simulink model "My_gfm_battery_sil_1_Exciter_1"  (R2018b)
settings: Solver=ode23t  StartTime=0.0  StopTime=30  MaxStep=1e-4  RelTol=1e-3
PreLoadFcn:
  | modelDir = fileparts(get_param(bdroot,'FileName'));
  | 
  | load_system(fullfile(modelDir,'controls_element_lib.slx'));
  | load_system(fullfile(modelDir,'test_sequence_lib.slx'));
InitFcn:
  | close all;
  | clear all;
  | clc;
  | 
  | % frequency nominals
  | F_NOM = 60;
  | W_NOM = 2 * pi * F_NOM;
  | 
  | % base values relative to inverter
  | % --------------------------------
  | VLL_INV_NOM = 480;
  | P_INV_NOM = 1e6;
  | Q_INV_NOM = 0.5e6;
  | S_INV_NOM = sqrt(P_INV_NOM^2 + Q_INV_NOM^2);
  | 
  | I_INV_BASE = S_INV_NOM/(sqrt(3)*VLL_INV_NOM);
  | Z_INV_BASE = VLL_INV_NOM^2/S_INV_NOM;
  | L_INV_BASE = Z_INV_BASE / W_NOM;
  | C_INV_BASE = 1 / (Z_INV_BASE * W_NOM);
  | 
  | % nominal ratings for power system model
  | % --------------------------------------
  | INVERTER_COUNT = 100;
  | 
  | VLV_NOM = VLL_INV_NOM;
  | VMV_NOM = 35e3;
  | VHV_NOM = 230e3;
  | S_PLANT = INVERTER_COUNT * S_INV_NOM;
  | 
  | N_GSU = VHV_NOM/VMV_NOM;
  | N_MVT = VMV_NOM/VLV_NOM;
  | 
  | I_LV_BASE = S_PLANT/(sqrt(3)*VLV_NOM);
  | I_MV_BASE = S_PLANT/(sqrt(3)*VMV_NOM);
  | I_HV_BASE = S_PLANT/(sqrt(3)*VHV_NOM);
  | 
  | Z_LV_BASE = VLV_NOM^2/S_PLANT;
  | Z_MV_BASE = VMV_NOM^2/S_PLANT;
  | Z_HV_BASE = VHV_NOM^2/S_PLANT;
  | 
  | L_LV_BASE = Z_LV_BASE / W_NOM;
  | L_MV_BASE = Z_MV_BASE / W_NOM;
  | L_HV_BASE = Z_HV_BASE / W_NOM;
  | C_LV_BASE = 1 / (Z_LV_BASE * W_NOM);
  | C_MV_BASE = 1 / (Z_MV_BASE * W_NOM);
  | C_HV_BASE = 1 / (Z_HV_BASE * W_NOM);
undefined symbols (not defined in the file): j
libraries: simulink x38, test_sequence_lib x10, controls_element_lib x9
(part 2 of 6)

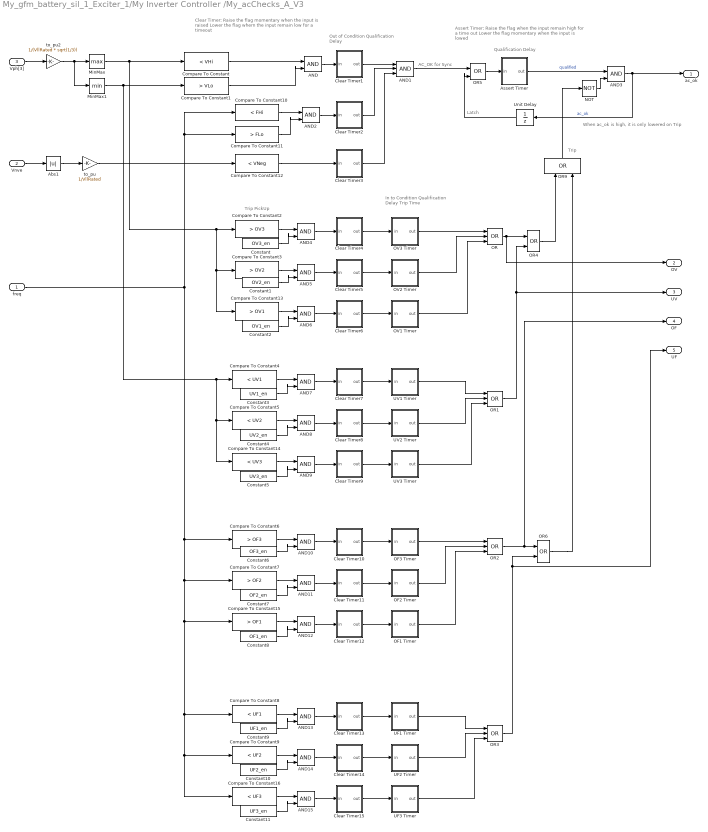
== system My_gfm_battery_sil_1_Exciter_1/My Inverter Controller /My_acChecks_A_V3 ==
  note: Trip
  note: Clear Timer:
      | Raise the flag momentary when the input is raised
      | Lower the flag whern the input remain low for a timeout
  note: AC_OK for Sync
  note: Assert Timer:
      | Raise the flag when the input remain high for a time out
      | Lower the flag momentary when the input is lowed
  note: Latch
  note: Qualification Delay
  note: When ac_ok is high, it is only lowered on Trip
  note: Out of Condition
      | Qualification Delay
  note: In to Condition
      | Qualification Delay
      | Trip Time
  note: Trip PickUp
  freq : Inport
  Vnve : Inport  Port=2
  Vph[3] : Inport  Port=3
  AND{,2..15} (15 alike) : Logic  IconShape=distinctive  AllPortsSameDT=off  OutDataTypeStr=boolean
  AND1 : Logic  Inputs=3  IconShape=distinctive  AllPortsSameDT=off  OutDataTypeStr=boolean
  Abs1 : Abs
  Assert Timer : Subsystem  mask{T_STEP=Ts, TIMEOUT=Time1}
      mask prompts: T_STEP "Time step"
  Clear Timer1 : Subsystem  mask{T_STEP=Ts, TIMEOUT=Time2, TIMER_INIT=0}
      mask prompts: T_STEP "Time step"; TIMER_INIT "Timer initial value"
  Clear Timer10 : Subsystem  mask{T_STEP=Ts, TIMEOUT=Time3, TIMER_INIT=0}
      mask prompts: T_STEP "Time step"; TIMER_INIT "Timer initial value"
  Clear Timer11 : Subsystem  mask{T_STEP=Ts, TIMEOUT=Time3, TIMER_INIT=0}
      mask prompts: T_STEP "Time step"; TIMER_INIT "Timer initial value"
  Clear Timer12 : Subsystem  mask{T_STEP=Ts, TIMEOUT=Time3, TIMER_INIT=0}
      mask prompts: T_STEP "Time step"; TIMER_INIT "Timer initial value"
  Clear Timer13 : Subsystem  mask{T_STEP=Ts, TIMEOUT=Time3, TIMER_INIT=0}
      mask prompts: T_STEP "Time step"; TIMER_INIT "Timer initial value"
  Clear Timer14 : Subsystem  mask{T_STEP=Ts, TIMEOUT=Time3, TIMER_INIT=0}
      mask prompts: T_STEP "Time step"; TIMER_INIT "Timer initial value"
  Clear Timer15 : Subsystem  mask{T_STEP=Ts, TIMEOUT=Time3, TIMER_INIT=0}
      mask prompts: T_STEP "Time step"; TIMER_INIT "Timer initial value"
  Clear Timer2 : Subsystem  mask{T_STEP=Ts, TIMEOUT=Time2, TIMER_INIT=0}
      mask prompts: T_STEP "Time step"; TIMER_INIT "Timer initial value"
  Clear Timer3 : Subsystem  mask{T_STEP=Ts, TIMEOUT=Time2, TIMER_INIT=0}
      mask prompts: T_STEP "Time step"; TIMER_INIT "Timer initial value"
  Clear Timer4 : Subsystem  mask{T_STEP=Ts, TIMEOUT=Time3, TIMER_INIT=0}
      mask prompts: T_STEP "Time step"; TIMER_INIT "Timer initial value"
  Clear Timer5 : Subsystem  mask{T_STEP=Ts, TIMEOUT=Time3, TIMER_INIT=0}
      mask prompts: T_STEP "Time step"; TIMER_INIT "Timer initial value"
  Clear Timer6 : Subsystem  mask{T_STEP=Ts, TIMEOUT=Time3, TIMER_INIT=0}
      mask prompts: T_STEP "Time step"; TIMER_INIT "Timer initial value"
  Clear Timer7 : Subsystem  mask{T_STEP=Ts, TIMEOUT=Time3, TIMER_INIT=0}
      mask prompts: T_STEP "Time step"; TIMER_INIT "Timer initial value"
  Clear Timer8 : Subsystem  mask{T_STEP=Ts, TIMEOUT=Time3, TIMER_INIT=0}
      mask prompts: T_STEP "Time step"; TIMER_INIT "Timer initial value"
  Clear Timer9 : Subsystem  mask{T_STEP=Ts, TIMEOUT=Time3, TIMER_INIT=0}
      mask prompts: T_STEP "Time step"; TIMER_INIT "Timer initial value"
  Compare To Constant : simulink/Logic and Bit Operations/Compare To Constant  relop=<  const=VHi  OutDataTypeStr=boolean
  Compare To Constant1 : simulink/Logic and Bit Operations/Compare To Constant  relop=>  const=VLo  OutDataTypeStr=boolean
  Compare To Constant10 : simulink/Logic and Bit Operations/Compare To Constant  relop=<  const=FHi  OutDataTypeStr=boolean
  Compare To Constant11 : simulink/Logic and Bit Operations/Compare To Constant  relop=>  const=FLo  OutDataTypeStr=boolean
  Compare To Constant12 : simulink/Logic and Bit Operations/Compare To Constant  relop=<  const=VNeg  OutDataTypeStr=boolean
  Compare To Constant13 : simulink/Logic and Bit Operations/Compare To Constant  relop=>  const=OV1  OutDataTypeStr=boolean
  Compare To Constant14 : simulink/Logic and Bit Operations/Compare To Constant  relop=<  const=UV3  OutDataTypeStr=boolean
  Compare To Constant15 : simulink/Logic and Bit Operations/Compare To Constant  relop=>  const=OF1  OutDataTypeStr=boolean
  Compare To Constant16 : simulink/Logic and Bit Operations/Compare To Constant  relop=<  const=UF3  OutDataTypeStr=boolean
  Compare To Constant2 : simulink/Logic and Bit Operations/Compare To Constant  relop=>  const=OV3  OutDataTypeStr=boolean
  Compare To Constant3 : simulink/Logic and Bit Operations/Compare To Constant  relop=>  const=OV2  OutDataTypeStr=boolean
  Compare To Constant4 : simulink/Logic and Bit Operations/Compare To Constant  relop=<  const=UV1  OutDataTypeStr=boolean
  Compare To Constant5 : simulink/Logic and Bit Operations/Compare To Constant  relop=<  const=UV2  OutDataTypeStr=boolean
  Compare To Constant6 : simulink/Logic and Bit Operations/Compare To Constant  relop=>  const=OF3  OutDataTypeStr=boolean
  Compare To Constant7 : simulink/Logic and Bit Operations/Compare To Constant  relop=>  const=OF2  OutDataTypeStr=boolean
  Compare To Constant8 : simulink/Logic and Bit Operations/Compare To Constant  relop=<  const=UF1  OutDataTypeStr=boolean
  Compare To Constant9 : simulink/Logic and Bit Operations/Compare To Constant  relop=<  const=UF2  OutDataTypeStr=boolean
  Constant : Constant  Value=OV3_en
  Constant1 : Constant  Value=OV2_en
  Constant10 : Constant  Value=UF2_en
  Constant11 : Constant  Value=UF3_en
  Constant2 : Constant  Value=OV1_en
  Constant3 : Constant  Value=UV1_en
  Constant4 : Constant  Value=UV2_en
  Constant5 : Constant  Value=UV3_en
  Constant6 : Constant  Value=OF3_en
  Constant7 : Constant  Value=OF2_en
  Constant8 : Constant  Value=OF1_en
  Constant9 : Constant  Value=UF1_en
  MinMax : MinMax  Function=max
  MinMax1 : MinMax
  NOT : Logic  Operator=NOT  IconShape=distinctive  AllPortsSameDT=off  OutDataTypeStr=boolean
  OF1 Timer : Subsystem  mask{T_STEP=Ts, TIMEOUT=OF1_Time}
      mask prompts: T_STEP "Time step"
  OF2 Timer : Subsystem  mask{T_STEP=Ts, TIMEOUT=OF2_Time}
      mask prompts: T_STEP "Time step"
  OF3 Timer : Subsystem  mask{T_STEP=Ts, TIMEOUT=OF3_Time}
      mask prompts: T_STEP "Time step"
  OR{,1..3} (4 alike) : Logic  Operator=OR  Inputs=3  IconShape=distinctive  AllPortsSameDT=off  OutDataTypeStr=boolean
  OR{4..6,9} (4 alike) : Logic  Operator=OR  IconShape=distinctive  AllPortsSameDT=off  OutDataTypeStr=boolean
  OV1 Timer : Subsystem  mask{T_STEP=Ts, TIMEOUT=OV1_Time}
      mask prompts: T_STEP "Time step"
  OV2 Timer : Subsystem  mask{T_STEP=Ts, TIMEOUT=OV2_Time}
      mask prompts: T_STEP "Time step"
  OV3 Timer : Subsystem  mask{T_STEP=Ts, TIMEOUT=OV3_Time}
      mask prompts: T_STEP "Time step"
  UF1 Timer : Subsystem  mask{T_STEP=Ts, TIMEOUT=UF1_Time}
      mask prompts: T_STEP "Time step"
  UF2 Timer : Subsystem  mask{T_STEP=Ts, TIMEOUT=UF2_Time}
      mask prompts: T_STEP "Time step"
  UF3 Timer : Subsystem  mask{T_STEP=Ts, TIMEOUT=UF3_Time}
      mask prompts: T_STEP "Time step"
  UV1 Timer : Subsystem  mask{T_STEP=Ts, TIMEOUT=UV1_Time}
      mask prompts: T_STEP "Time step"
  UV2 Timer : Subsystem  mask{T_STEP=Ts, TIMEOUT=UV2_Time}
      mask prompts: T_STEP "Time step"
  UV3 Timer : Subsystem  mask{T_STEP=Ts, TIMEOUT=UV3_Time}
      mask prompts: T_STEP "Time step"
  Unit Delay : UnitDelay  SampleTime=Ts
  to_pu : Gain  Gain=1/VllRated
  to_pu2 : Gain  Gain=1/(VllRated * sqrt(1/3))
  ac_ok : Outport  VectorParamsAs1DForOutWhenUnconnected=on
  OV : Outport  Port=2  VectorParamsAs1DForOutWhenUnconnected=on
  UV : Outport  Port=3  VectorParamsAs1DForOutWhenUnconnected=on
  OF : Outport  Port=4  VectorParamsAs1DForOutWhenUnconnected=on
  UF : Outport  Port=5  VectorParamsAs1DForOutWhenUnconnected=on
  wires:
  Vph[3]/1 -> to_pu2/1
  OR4/1 -> OR9/1
  OR9/1 -> NOT/1
  to_pu/1 -> Compare To Constant12/1
  MinMax/1 -> Compare To Constant13/1, Compare To Constant3/1, Compare To Constant2/1, Compare To Constant/1
  Abs1/1 -> to_pu/1
  Unit Delay/1 -> OR5/2
  OV3 Timer/1(out) -> OR/1
  Compare To Constant12/1 -> Clear Timer3/1(in)
  Clear Timer3/1(out) -> AND1/3
  Assert Timer/1(out) -> AND3/1  "qualified"
  UV2 Timer/1(out) -> OR1/2
  OF3 Timer/1(out) -> OR2/1
  Clear Timer10/1(out) -> OF3 Timer/1(in)
  Compare To Constant6/1 -> AND10/1
  Clear Timer11/1(out) -> OF2 Timer/1(in)
  Clear Timer4/1(out) -> OV3 Timer/1(in)
  UF1 Timer/1(out) -> OR3/1
  UF2 Timer/1(out) -> OR3/2
  Vnve/1 -> Abs1/1
  NOT/1 -> AND3/2
  UV1 Timer/1(out) -> OR1/1
  AND2/1 -> Clear Timer2/1(in)
  Compare To Constant11/1 -> AND2/2
  OF2 Timer/1(out) -> OR2/2
  Clear Timer7/1(out) -> UV1 Timer/1(in)
  OR1/1 -> UV/1, OR4/2
  Clear Timer13/1(out) -> UF1 Timer/1(in)
  Compare To Constant7/1 -> AND11/1
  Clear Timer2/1(out) -> AND1/2
  Clear Timer14/1(out) -> UF2 Timer/1(in)
  Clear Timer5/1(out) -> OV2 Timer/1(in)
  freq/1 -> Compare To Constant11/1, Compare To Constant10/1, Compare To Constant8/1, Compare To Constant16/1, Compare To Constant9/1, Compare To Constant15/1, Compare To Constant7/1, Compare To Constant6/1
  OV2 Timer/1(out) -> OR/2
  Compare To Constant10/1 -> AND2/1
  Clear Timer1/1(out) -> AND1/1
  OR/1 -> OV/1, OR4/1
  Clear Timer8/1(out) -> UV2 Timer/1(in)
  AND3/1 -> ac_ok/1, Unit Delay/1  "ac_ok"
  Compare To Constant2/1 -> AND4/1
  Compare To Constant3/1 -> AND5/1
  AND/1 -> Clear Timer1/1(in)
  Compare To Constant/1 -> AND/1
  Compare To Constant1/1 -> AND/2
  AND1/1 -> OR5/1
  OR5/1 -> Assert Timer/1(in)
  to_pu2/1 -> MinMax1/1, MinMax/1
  Clear Timer6/1(out) -> OV1 Timer/1(in)
  OV1 Timer/1(out) -> OR/3
  Clear Timer9/1(out) -> UV3 Timer/1(in)
  UV3 Timer/1(out) -> OR1/3
  MinMax1/1 -> Compare To Constant4/1, Compare To Constant14/1, Compare To Constant5/1, Compare To Constant1/1
  Compare To Constant15/1 -> AND12/1
  OF1 Timer/1(out) -> OR2/3
  Clear Timer12/1(out) -> OF1 Timer/1(in)
  Clear Timer15/1(out) -> UF3 Timer/1(in)
  UF3 Timer/1(out) -> OR3/3
  AND4/1 -> Clear Timer4/1(in)
  Constant/1 -> AND4/2
  AND5/1 -> Clear Timer5/1(in)
  Constant1/1 -> AND5/2
  Compare To Constant13/1 -> AND6/1
  AND6/1 -> Clear Timer6/1(in)
  Constant2/1 -> AND6/2
  Compare To Constant4/1 -> AND7/1
  AND7/1 -> Clear Timer7/1(in)
  Compare To Constant5/1 -> AND8/1
  AND8/1 -> Clear Timer8/1(in)
  Compare To Constant14/1 -> AND9/1
  AND9/1 -> Clear Timer9/1(in)
  Constant3/1 -> AND7/2
  Constant4/1 -> AND8/2
  Constant5/1 -> AND9/2
  AND10/1 -> Clear Timer10/1(in)
  AND11/1 -> Clear Timer11/1(in)
  AND12/1 -> Clear Timer12/1(in)
  Constant6/1 -> AND10/2
  Constant7/1 -> AND11/2
  Constant8/1 -> AND12/2
  Compare To Constant8/1 -> AND13/1
  Constant9/1 -> AND13/2
  Compare To Constant9/1 -> AND14/1
  Constant10/1 -> AND14/2
  AND13/1 -> Clear Timer13/1(in)
  AND14/1 -> Clear Timer14/1(in)
  AND15/1 -> Clear Timer15/1(in)
  Compare To Constant16/1 -> AND15/1
  Constant11/1 -> AND15/2
  OR2/1 -> OF/1, OR6/1
  OR3/1 -> OR6/2, UF/1
  OR6/1 -> OR9/2

== system My_gfm_battery_sil_1_Exciter_1/My Inverter Controller /My_acMonitor_A ==
  note: Remove the second order ripple, dc value is RMS
  note: RMS LL Pos Seq Voltage (Vd+, Vq+)
  note: RMS LL Neg Seq Voltage (Vd-, Vq-)
  note: cos x + j sin x
      | cos (x-120) + j (sin x -120)
      | cos (x+120) + j (sin x +120)
  note: Hz
  note: RMS Va, Vb, Vc
  v_ac : Inport
  Analyzer_V : Subsystem
  Analyzer_V1 : Subsystem  Commented=on
  Gain2 : Gain  Gain=2
  PLL_3ph : Subsystem
  RMS_Analyzer : Subsystem
  SOGI : Subsystem
  Scope : Scope  NumInputPorts=3
  Scope1 : Scope  NumInputPorts=4
  Scope2 : Scope  NumInputPorts=2
  Terminator : Terminator
  to_pu : Gain  Gain=1/VllRated
  pll_freq : Outport  VectorParamsAs1DForOutWhenUnconnected=on
  pll_osc[3] : Outport  Port=2  VectorParamsAs1DForOutWhenUnconnected=on
  Vpve : Outport  Port=3  VectorParamsAs1DForOutWhenUnconnected=on
  Vnve : Outport  Port=4  VectorParamsAs1DForOutWhenUnconnected=on
  Vph[3] : Outport  Port=5  VectorParamsAs1DForOutWhenUnconnected=on
  wires:
  SOGI/1(notch) -> Scope/3, Vph[3]/1
  Gain2/1 -> SOGI/2(fnom)
  RMS_Analyzer/1(RMS) -> Scope/2, SOGI/1(in)
  Analyzer_V/4(Nve) -> Scope1/4, Vnve/1
  Analyzer_V/3(Pve) -> Vpve/1, Scope1/3
  PLL_3ph/1(osc[3]) -> pll_osc[3]/1, Scope2/2, Analyzer_V/2(osc[3])
  PLL_3ph/2(freq) -> Gain2/1, pll_freq/1
  v_ac/1 -> to_pu/1, Analyzer_V/1(in[3]), Scope/1, RMS_Analyzer/1(in)
  to_pu/1 -> Scope2/1, PLL_3ph/1(ref)
  Analyzer_V/1(fund[3]) -> Scope1/1
  Analyzer_V/2(Zero) -> Scope1/2
  SOGI/2(bpf) -> Terminator/1

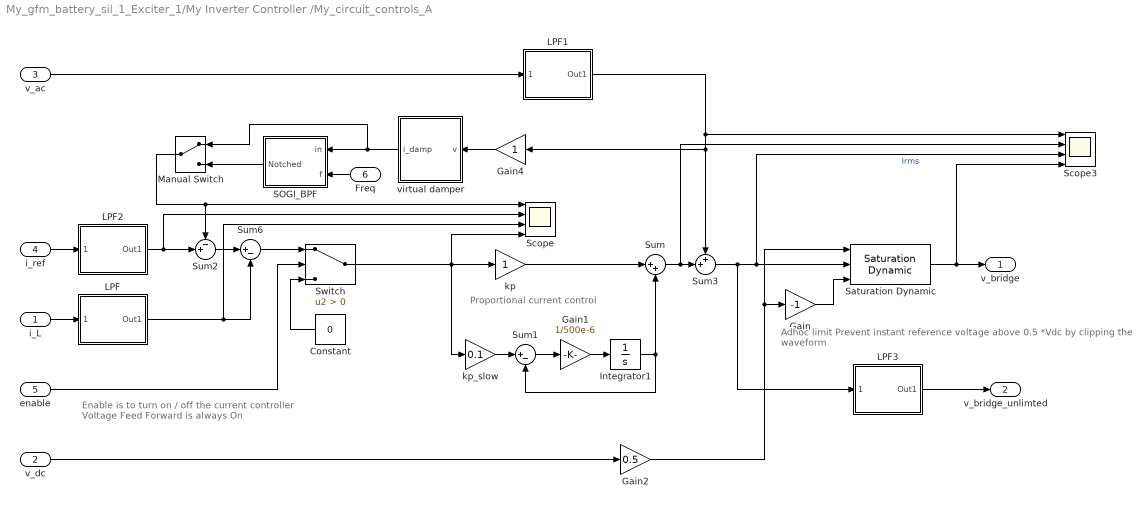
== system My_gfm_battery_sil_1_Exciter_1/My Inverter Controller /My_circuit_controls_A ==
  note: Proportional current control
  note: Adhoc limit
      | Prevent instant reference voltage above 0.5 *Vdc by clipping the waveform
  note: Enable is to turn on / off the current controller
      | Voltage Feed Forward is always On
  i_L : Inport
  v_dc : Inport  Port=2
  v_ac : Inport  Port=3
  i_ref : Inport  Port=4
  enable : Inport  Port=5
  Freq : Inport  Port=6
  Constant : Constant  Value=0
  Gain : Gain  Gain=-1
  Gain1 : Gain  Gain=1/500e-6
  Gain2 : Gain  Gain=0.5
  Gain4 : Gain
  Integrator1 : Integrator
  LPF : Subsystem
  LPF1 : Subsystem
  LPF2 : Subsystem
  LPF3 : Subsystem
  Manual Switch : ManualSwitch
  SOGI_BPF : Subsystem
  Saturation Dynamic : simulink/Discontinuities/Saturation Dynamic  OutMin=[]  OutMax=[]  OutDataTypeStr=Inherit: Same as second input  OutDataType=fixdt(1, 16)  OutScaling=2^-10  DoSatur=off
  Scope : Scope  NumInputPorts=4
  Scope3 : Scope  NumInputPorts=4
  Sum : Sum  Inputs=|++
  Sum1 : Sum  Inputs=|+-
  Sum2 : Sum  Inputs=-+|
  Sum3 : Sum  Inputs=++|
  Sum6 : Sum  Inputs=|+-
  Switch : Switch  Criteria=u2 > Threshold
  kp : Gain
  kp_slow : Gain  Gain=0.1
  virtual damper : Subsystem
  v_bridge : Outport  VectorParamsAs1DForOutWhenUnconnected=on
  v_bridge_unlimted : Outport  Port=2  VectorParamsAs1DForOutWhenUnconnected=on
  wires:
  LPF1/1(Out1) -> Gain4/1, Sum3/1, Scope3/1
  LPF/1(Out1) -> Scope/3, Sum6/2
  Gain2/1 -> Gain/1, Saturation Dynamic/1
  v_ac/1 -> LPF1/1(1)
  enable/1 -> Switch/2
  Constant/1 -> Switch/3
  Sum6/1 -> Switch/1
  i_ref/1 -> LPF2/1(1)
  i_L/1 -> LPF/1(1)
  Saturation Dynamic/1 -> Scope3/4, v_bridge/1
  Sum/1 -> Scope3/2, Sum3/2
  Sum2/1 -> Sum6/1
  kp/1 -> Sum/1
  Integrator1/1 -> Sum/2, Sum1/2
  Sum1/1 -> Gain1/1
  Gain1/1 -> Integrator1/1
  kp_slow/1 -> Sum1/1
  v_dc/1 -> Gain2/1
  Gain/1 -> Saturation Dynamic/3
  LPF2/1(Out1) -> Scope/2, Sum2/2
  Switch/1 -> Scope/4, kp/1, kp_slow/1
  Gain4/1 -> virtual damper/1(v)
  Freq/1 -> SOGI_BPF/2(f)
  virtual damper/1(i_damp) -> Manual Switch/1, SOGI_BPF/1(in)
  Manual Switch/1 -> Scope/1, Sum2/1
  SOGI_BPF/1(Notched) -> Manual Switch/2
  Sum3/1 -> LPF3/1(1), Scope3/3, Saturation Dynamic/2  "Irms"
  LPF3/1(Out1) -> v_bridge_unlimted/1

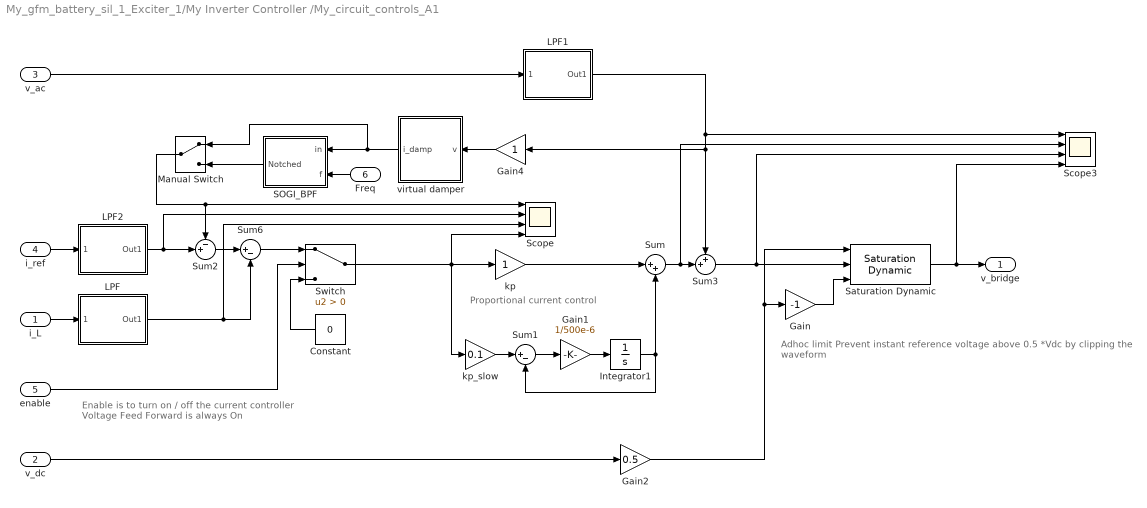
== system My_gfm_battery_sil_1_Exciter_1/My Inverter Controller /My_circuit_controls_A1 ==
  note: Proportional current control
  note: Adhoc limit
      | Prevent instant reference voltage above 0.5 *Vdc by clipping the waveform
  note: Enable is to turn on / off the current controller
      | Voltage Feed Forward is always On
  i_L : Inport
  v_dc : Inport  Port=2
  v_ac : Inport  Port=3
  i_ref : Inport  Port=4
  enable : Inport  Port=5
  Freq : Inport  Port=6
  Constant : Constant  Value=0
  Gain : Gain  Gain=-1
  Gain1 : Gain  Gain=1/500e-6
  Gain2 : Gain  Gain=0.5
  Gain4 : Gain
  Integrator1 : Integrator
  LPF : Subsystem
  LPF1 : Subsystem
  LPF2 : Subsystem
  Manual Switch : ManualSwitch
  SOGI_BPF : Subsystem
  Saturation Dynamic : simulink/Discontinuities/Saturation Dynamic  OutMin=[]  OutMax=[]  OutDataTypeStr=Inherit: Same as second input  OutDataType=fixdt(1, 16)  OutScaling=2^-10  DoSatur=off
  Scope : Scope  NumInputPorts=4
  Scope3 : Scope  NumInputPorts=4
  Sum : Sum  Inputs=|++
  Sum1 : Sum  Inputs=|+-
  Sum2 : Sum  Inputs=-+|
  Sum3 : Sum  Inputs=++|
  Sum6 : Sum  Inputs=|+-
  Switch : Switch  Criteria=u2 > Threshold
  kp : Gain
  kp_slow : Gain  Gain=0.1
  virtual damper : Subsystem
  v_bridge : Outport  VectorParamsAs1DForOutWhenUnconnected=on
  wires:
  LPF1/1(Out1) -> Gain4/1, Sum3/1, Scope3/1
  LPF/1(Out1) -> Scope/3, Sum6/2
  Gain2/1 -> Gain/1, Saturation Dynamic/1
  v_ac/1 -> LPF1/1(1)
  enable/1 -> Switch/2
  Constant/1 -> Switch/3
  Sum6/1 -> Switch/1
  Sum3/1 -> Scope3/3, Saturation Dynamic/2
  i_ref/1 -> LPF2/1(1)
  i_L/1 -> LPF/1(1)
  Saturation Dynamic/1 -> Scope3/4, v_bridge/1
  Sum/1 -> Scope3/2, Sum3/2
  Sum2/1 -> Sum6/1
  kp/1 -> Sum/1
  Integrator1/1 -> Sum/2, Sum1/2
  Sum1/1 -> Gain1/1
  Gain1/1 -> Integrator1/1
  kp_slow/1 -> Sum1/1
  v_dc/1 -> Gain2/1
  Gain/1 -> Saturation Dynamic/3
  LPF2/1(Out1) -> Scope/2, Sum2/2
  Switch/1 -> Scope/4, kp/1, kp_slow/1
  Gain4/1 -> virtual damper/1(v)
  Freq/1 -> SOGI_BPF/2(f)
  virtual damper/1(i_damp) -> Manual Switch/1, SOGI_BPF/1(in)
  Manual Switch/1 -> Scope/1, Sum2/1
  SOGI_BPF/1(Notched) -> Manual Switch/2

== system My_gfm_battery_sil_1_Exciter_1/My Inverter Controller /My_currentLimiting_B ==
  note: LL RMS
  note: SOGI gain is 1 not 1/sqrt(2),
      | improve tracking over transients
  note: Only capture 60Hz component
  note: Iabc rms
  note: Peak_Iabc
  note: Only apply limit on 60 Hz components
  note: LL RMS
  Irms_limit : Inport
  freq : Inport  Port=2
  iref : Inport  Port=3
  v_bridge_unlimted : Inport  Port=4
  v_dc : Inport  Port=5
  Constant1 : Constant
  Current_foldback1 : Subsystem
  Gain1 : Gain  Gain=sqrt(3/2)
  Gain2 : Gain  Gain=0.5
  Gain3 : Gain  Gain=sqrt(3)
  Manual Switch : ManualSwitch  CurrentSetting=0
  Product : Product
  Product1 : Product
  RMS_Analyzer : Subsystem
  RMS_Analyzer1 : Subsystem
  SOGI_BPF : Subsystem
  Scope1 : Scope  NumInputPorts=3
  Scope11 : Scope  NumInputPorts=3
  Scope3 : Scope  NumInputPorts=3
  Sum1 : Sum  Inputs=|+-
  estimate_excess : Subsystem
  soft_saturation : Subsystem  mask{soft_limit=peakSoftLimit*IRated, hard_limit=peakHardLimit*IRated, Xau=1}
      mask prompts: soft_limit "Soft limit"; hard_limit "Hard limit"; Xau "Saturation Rate"
  soft_saturation1 : Subsystem  Commented=on  mask{soft_limit=peakSoftLimit*IRated, hard_limit=peakHardLimit*IRated}
      mask prompts: soft_limit "Soft limit"; hard_limit "Hard limit"
  to_pu : Gain  Gain=1/VLL_INV_NOM
  to_pu1 : Gain  Gain=1/VLL_INV_NOM
  iref_limited : Outport  VectorParamsAs1DForOutWhenUnconnected=on
  wires:
  soft_saturation/1(out) -> Scope3/2, Product/1
  estimate_excess/1(excess_fraction) -> Scope11/1, Product1/1
  RMS_Analyzer/1(RMS) -> estimate_excess/2(I[3])  "Irms"
  Product1/1 -> Scope11/3, Sum1/2  "i_excess"
  SOGI_BPF/1(bpf) -> Product1/2, Scope11/2
  freq/1 -> SOGI_BPF/2(f)
  iref/1 -> Sum1/1, RMS_Analyzer/1(in), SOGI_BPF/1(in)
  Irms_limit/1 -> estimate_excess/1(Ilimit)
  v_bridge_unlimted/1 -> RMS_Analyzer1/1(in)
  Sum1/1 -> soft_saturation/1(in)
  RMS_Analyzer1/1(RMS) -> Gain3/1
  v_dc/1 -> Gain2/1
  Gain2/1 -> Gain1/1
  to_pu/1 -> Current_foldback1/1(V[3]_pu), Scope1/2
  Gain3/1 -> to_pu/1
  to_pu1/1 -> Current_foldback1/2(Vmax), Scope1/3
  Product/1 -> Scope3/1, iref_limited/1
  Manual Switch/1 -> Product/2, Scope3/3
  Current_foldback1/1(limit_pu) -> Scope1/1, Manual Switch/2
  Constant1/1 -> Manual Switch/1
  Gain1/1 -> to_pu1/1

== system My_gfm_battery_sil_1_Exciter_1/My Inverter Controller /My_currentLimiting_B1 ==
  note: SOGI gain is 1 not 1/sqrt(2),
      | improve tracking over transients
  note: Only capture 60Hz component
  note: Iabc rms
  note: Peak_Iabc
  note: Only apply limit on 60 Hz components
  Irms_limit : Inport
  freq : Inport  Port=2
  iref : Inport  Port=3
  Product1 : Product
  RMS_Analyzer : Subsystem
  SOGI_BPF : Subsystem
  Scope11 : Scope  NumInputPorts=3
  Sum1 : Sum  Inputs=|+-
  estimate_excess : Subsystem
  soft_saturation : Subsystem  mask{soft_limit=peakSoftLimit*IRated, hard_limit=peakHardLimit*IRated, Xau=1}
      mask prompts: soft_limit "Soft limit"; hard_limit "Hard limit"; Xau "Saturation Rate"
  soft_saturation1 : Subsystem  Commented=on  mask{soft_limit=peakSoftLimit*IRated, hard_limit=peakHardLimit*IRated}
      mask prompts: soft_limit "Soft limit"; hard_limit "Hard limit"
  iref_limited : Outport  VectorParamsAs1DForOutWhenUnconnected=on
  wires:
  soft_saturation/1(out) -> iref_limited/1
  estimate_excess/1(excess_fraction) -> Scope11/1, Product1/1
  RMS_Analyzer/1(RMS) -> estimate_excess/2(I[3])  "Irms"
  Product1/1 -> Scope11/3, Sum1/2  "i_excess"
  Sum1/1 -> soft_saturation/1(in)
  SOGI_BPF/1(bpf) -> Product1/2, Scope11/2
  freq/1 -> SOGI_BPF/2(f)
  iref/1 -> Sum1/1, RMS_Analyzer/1(in), SOGI_BPF/1(in)
  Irms_limit/1 -> estimate_excess/1(Ilimit)

== system My_gfm_battery_sil_1_Exciter_1/My Inverter Controller /My_currentSource_A ==
  note: S = sqrt(3)*V *conj(I)
      | P+jQ = sqrt(3)*(vd+jvq)*(id-jiq)
      | so P-jQ = sqrt(3)*(vd-jvq)*(id+jiq)
      | vq = 0, vd is LL RMS, id,iq are RMS
  note: S = sqrt(3) * VLL_rms * Irms
  note: RMS Id, Iq
  note: Vd+
  note: Why?
  note: RMS LL Pos Seq Voltage (Vd+, Vq+)
  note: Peak_Iabc
  note: cos x + j sin x
      | cos (x-120) + j (sin x -120)
      | cos (x+120) + j (sin x +120)
  enable : Inport
  P_request : Inport  Port=2
  Q_request : Inport  Port=3
  osc : Inport  Port=4
  Vpve : Inport  Port=5
  AND4 : Logic  IconShape=distinctive  AllPortsSameDT=off  OutDataTypeStr=boolean
  Complex to Real-Imag : ComplexToRealImag
  Conj : Math  Operator=conj  SaturateOnIntegerOverflow=on
  Constant : Constant  Value=0
  Constant2 : Constant  Value=CSOnline
  Divide : Product  Inputs=*/
  Gain : Gain  Gain=1/sqrt(3)
  Max1 : MinMax  Function=max  Inputs=2
  Real-Imag to Complex : RealImagToComplex
  Scope : Scope
  Switch : Switch  Criteria=u2 > Threshold
  Terminator : Terminator
  VLL_RATED : Constant  Value=VllRated
  current_modulator : Subsystem
  iref : Outport  VectorParamsAs1DForOutWhenUnconnected=on
  wires:
  Q_request/1 -> Real-Imag to Complex/2
  P_request/1 -> Real-Imag to Complex/1
  Complex to Real-Imag/1 -> Max1/1
  VLL_RATED/1 -> Max1/2
  Max1/1 -> Divide/2
  Divide/1 -> Gain/1
  Vpve/1 -> Complex to Real-Imag/1
  current_modulator/1(i_ref) -> Switch/1
  osc/1 -> current_modulator/2(osc)
  Real-Imag to Complex/1 -> Conj/1
  Conj/1 -> Divide/1
  Gain/1 -> Scope/1, current_modulator/1(I_cmd)
  Complex to Real-Imag/2 -> Terminator/1
  Constant/1 -> Switch/3
  Switch/1 -> iref/1
  Constant2/1 -> AND4/2
  AND4/1 -> Switch/2
  enable/1 -> AND4/1

== system My_gfm_battery_sil_1_Exciter_1/My Inverter Controller /My_machineModel_A ==
  note: Assume circuit controls will achieve
      | Iref = Imeas in the freq range of interest
  note: Measured terminal voltage
  note: Aligning with Rotor Frame
      | cos x + j sin x
      | cos (x-120) + j (sin x -120)
      | cos (x+120) + j (sin x +120)
  note: Peak Va, Vb, Vc
  note: RMS LL Vd
  note: RMS LL Vq
  Vref : Inport
  Prequest : Inport  Port=2
  Ex_Fref : Inport  Port=3
  PLL_Fref : Inport  Port=4
  v_terminal : Inport  Port=5
  enable : Inport  Port=6
  AND4 : Logic  IconShape=distinctive  AllPortsSameDT=off  OutDataTypeStr=boolean
  AVR : Subsystem  AncestorBlock=controls_element_lib/machineModel_A/excitation
  Constant1 : Constant  Value=FreqRefSel
  Constant2 : Constant  Value=MachOnline
  Exciter : Subsystem  AncestorBlock=controls_element_lib/machineModel_A/excitation
  Scope : Scope  NumInputPorts=3
  Scope1 : Scope  NumInputPorts=4
  Scope2 : Scope  NumInputPorts=4
  Switch : Switch  Criteria=u2 > Threshold
  governer : Subsystem
  impedance emulation : Subsystem
  power analyzer : Subsystem
  rotor model : Subsystem
  voltage analyzer : Subsystem
  rotor_freq : Outport  VectorParamsAs1DForOutWhenUnconnected=on
  iref : Outport  Port=2  VectorParamsAs1DForOutWhenUnconnected=on
  wires:
  Vref/1 -> AVR/1(VRef)
  Switch/1 -> governer/2(Fref)
  AND4/1 -> governer/3(enabled), AVR/3(enabled), impedance emulation/2(enable)
  voltage analyzer/1(Vd) -> Scope2/2, AVR/6(Vd)
  rotor model/2(f_rotor) -> Scope1/4, governer/6(f_rotor), Scope/1, rotor_freq/1  "f_rotor"
  voltage analyzer/2(Vq) -> governer/5(Vq), Scope2/3, AVR/7(Vq)
  v_terminal/1 -> Scope2/1, voltage analyzer/2(v_terminal), power analyzer/2(vac), Scope/3, impedance emulation/3(v_terminal)
  impedance emulation/1(i_ref) -> iref/1, AVR/5(iac), power analyzer/1(iac)
  Prequest/1 -> governer/1(Prequest)
  governer/1(power) -> Scope1/1, rotor model/1(p_mechanical)
  Exciter/1(v_emf) -> Scope/2, impedance emulation/1(v_emf)  "v_emf"
  power analyzer/1(P) -> Scope1/2, rotor model/2(p_electrical)  "p_electrical"
  rotor model/1(osc[3]) -> voltage analyzer/1(osc[3]), Exciter/2(osc[3]), AVR/4(osc[3])
  power analyzer/2(Q) -> Scope1/3, AVR/2(Q)
  voltage analyzer/3(Vt_Mag) -> governer/4(Vt), Scope2/4
  Constant1/1 -> Switch/2
  Ex_Fref/1 -> Switch/1
  PLL_Fref/1 -> Switch/3
  Constant2/1 -> AND4/2
  enable/1 -> AND4/1
  AVR/1(Vexc) -> Exciter/1(Vexc)

== system My_gfm_battery_sil_1_Exciter_1/My Inverter Controller /My_machineModel_A1 ==
  note: Assume circuit controls will achieve
      | Iref = Imeas in the freq range of interest
  note: Measured terminal voltage
  note: Aligning with Rotor Frame
      | cos x + j sin x
      | cos (x-120) + j (sin x -120)
      | cos (x+120) + j (sin x +120)
  note: Peak Va, Vb, Vc
  note: RMS LL Vd
  note: RMS LL Vq
  Vref : Inport
  Prequest : Inport  Port=2
  Ex_Fref : Inport  Port=3
  PLL_Fref : Inport  Port=4
  v_terminal : Inport  Port=5
  enable : Inport  Port=6
  AND4 : Logic  IconShape=distinctive  AllPortsSameDT=off  OutDataTypeStr=boolean
  Constant1 : Constant  Value=FreqRefSel
  Constant2 : Constant  Value=MachOnline
  Scope : Scope  NumInputPorts=3
  Scope1 : Scope  NumInputPorts=4
  Scope2 : Scope  NumInputPorts=4
  Switch : Switch  Criteria=u2 > Threshold
  Terminator : Terminator
  excitation : Subsystem  AncestorBlock=controls_element_lib/machineModel_A/excitation
  governer : Subsystem
  governer1 : Subsystem  Commented=on
  impedance emulation : Subsystem
  power analyzer : Subsystem
  rotor model : Subsystem
  voltage analyzer : Subsystem
  rotor_freq : Outport  VectorParamsAs1DForOutWhenUnconnected=on
  iref : Outport  Port=2  VectorParamsAs1DForOutWhenUnconnected=on
  wires:
  Vref/1 -> excitation/1(VRef)
  Switch/1 -> governer/2(Fref)
  AND4/1 -> governer/3(enabled), impedance emulation/2(enable)
  voltage analyzer/1(Vd) -> Scope2/2
  rotor model/2(f_rotor) -> Scope1/4, governer/6(f_rotor), Scope/1, rotor_freq/1  "f_rotor"
  voltage analyzer/2(Vq) -> governer/5(Vq), Scope2/3
  v_terminal/1 -> Scope2/1, voltage analyzer/2(v_terminal), power analyzer/2(vac), Scope/3, impedance emulation/3(v_terminal)
  impedance emulation/1(i_ref) -> iref/1, power analyzer/1(iac)
  Prequest/1 -> governer/1(Prequest)
  governer/1(power) -> Scope1/1, rotor model/1(p_mechanical)
  excitation/1(v_emf) -> Scope/2, impedance emulation/1(v_emf)  "v_emf"
  power analyzer/1(P) -> Scope1/2, rotor model/2(p_electrical)  "p_electrical"
  rotor model/1(osc[3]) -> excitation/2(osc[3]), voltage analyzer/1(osc[3])
  power analyzer/2(Q) -> Scope1/3, Terminator/1
  voltage analyzer/3(Vt_Mag) -> excitation/3(Vt), governer/4(Vt), Scope2/4
  Constant1/1 -> Switch/2
  Ex_Fref/1 -> Switch/1
  PLL_Fref/1 -> Switch/3
  Constant2/1 -> AND4/2
  enable/1 -> AND4/1

== system My_gfm_battery_sil_1_Exciter_1/My Inverter Controller /My_machineModel_Other Exciter ==
  note: Assume circuit controls will achieve
      | Iref = Imeas in the freq range of interest
  note: Measured terminal voltage
  note: Aligning with Rotor Frame
      | cos x + j sin x
      | cos (x-120) + j (sin x -120)
      | cos (x+120) + j (sin x +120)
  note: Peak Va, Vb, Vc
  note: RMS LL Vd
  note: RMS LL Vq
  Ex_Vref : Inport
  Prequest : Inport  Port=2
  Ex_Fref : Inport  Port=3
  PLL_Fref : Inport  Port=4
  v_terminal : Inport  Port=5
  enable : Inport  Port=6
  AND4 : Logic  IconShape=distinctive  AllPortsSameDT=off  OutDataTypeStr=boolean
  AVR : Subsystem  AncestorBlock=controls_element_lib/machineModel_A/excitation
  Constant1 : Constant  Value=FreqRefSel
  Constant2 : Constant  Value=MachOnline
  Exciter : Subsystem  AncestorBlock=controls_element_lib/machineModel_A/excitation
  Scope : Scope  NumInputPorts=3
  Scope1 : Scope  NumInputPorts=4
  Scope2 : Scope  NumInputPorts=4
  Switch : Switch  Criteria=u2 > Threshold
  governer : Subsystem
  impedance emulation : Subsystem
  power analyzer : Subsystem
  rotor model : Subsystem
  voltage analyzer : Subsystem
  rotor_freq : Outport  VectorParamsAs1DForOutWhenUnconnected=on
  iref : Outport  Port=2  VectorParamsAs1DForOutWhenUnconnected=on
  wires:
  Switch/1 -> governer/2(Fref)
  AND4/1 -> governer/3(enabled), impedance emulation/2(enable)
  voltage analyzer/1(Vd) -> AVR/2(Vt), Scope2/2
  rotor model/2(f_rotor) -> Scope1/4, governer/6(f_rotor), Scope/1, rotor_freq/1  "f_rotor"
  voltage analyzer/2(Vq) -> governer/5(Vq), Scope2/3
  v_terminal/1 -> Scope2/1, voltage analyzer/2(v_terminal), power analyzer/2(vac), Scope/3, impedance emulation/3(v_terminal)
  impedance emulation/1(i_ref) -> iref/1, power analyzer/1(iac)
  Prequest/1 -> governer/1(Prequest)
  governer/1(power) -> Scope1/1, rotor model/1(p_mechanical)
  Exciter/1(v_emf) -> Scope/2, impedance emulation/1(v_emf)  "v_emf"
  power analyzer/1(P) -> Scope1/2, rotor model/2(p_electrical)  "p_electrical"
  rotor model/1(osc[3]) -> voltage analyzer/1(osc[3]), Exciter/2(osc[3])
  power analyzer/2(Q) -> AVR/3(Q), Scope1/3
  voltage analyzer/3(Vt_Mag) -> governer/4(Vt), Scope2/4
  Constant1/1 -> Switch/2
  Ex_Fref/1 -> Switch/1
  PLL_Fref/1 -> Switch/3
  Constant2/1 -> AND4/2
  enable/1 -> AND4/1
  AVR/1(Vexc) -> Exciter/1(Vexc)
  Ex_Vref/1 -> AVR/1(VRef)

== system My_gfm_battery_sil_1_Exciter_1/My Inverter Controller /My_powerLimiter_A ==
  note: Why not using Vpve
  note: RMS_Id
  note: Peak_Iabc
  note: Power Limits from Battery Management system
  note: Ref current (Machine + Current source)
  note: cos x + j sin x
      | cos (x-120) + j (sin x -120)
      | cos (x+120) + j (sin x +120)
  i_ac : Inport
  v_ac : Inport  Port=2
  osc : Inport  Port=3
  P_lim_high : Inport  Port=4
  P_lim_low : Inport  Port=5
  Gain1 : Gain  Gain=1/(VllRated * sqrt(3))
  Product : Product
  Saturation Dynamic : simulink/Discontinuities/Saturation Dynamic  OutMin=[]  OutMax=[]  OutDataTypeStr=Inherit: Same as second input  OutDataType=fixdt(1, 16)  OutScaling=2^-10  DoSatur=off
  Sum of Elements : Sum  Inputs=+
  Sum1 : Sum  Inputs=|+-
  Transfer Fcn : TransferFcn  Denominator=[1/wPowerLimiter, 1]
  current_modulator : controls_element_lib/currentSource_A/current_modulator  SystemSampleTime=-1
  i_excess : Outport  VectorParamsAs1DForOutWhenUnconnected=on
  wires:
  Transfer Fcn/1 -> Sum1/1, Saturation Dynamic/2  "P_lpf"
  current_modulator/1 -> i_excess/1
  Saturation Dynamic/1 -> Sum1/2
  P_lim_low/1 -> Saturation Dynamic/3
  P_lim_high/1 -> Saturation Dynamic/1
  Sum1/1 -> Gain1/1
  Sum of Elements/1 -> Transfer Fcn/1  "P_inst"
  Gain1/1 -> current_modulator/1
  osc/1 -> current_modulator/2
  Product/1 -> Sum of Elements/1
  i_ac/1 -> Product/1
  v_ac/1 -> Product/2

== system My_gfm_battery_sil_1_Exciter_1/Plant controller (simplified example)/LVRT_foldback ==
  note: Delay the Power ramping after voltage drop
  Vpve_pu : Inport
  Complex to Magnitude-Angle : ComplexToMagnitudeAngle
  Constant1 : Constant
  Gain : Gain  Gain=5
  LPF : Subsystem
  Saturation : Saturate  UpperLimit=1  LowerLimit=0.05
  Sum1 : Sum  Inputs=|+-
  Sum2 : Sum  Inputs=|++
  Terminator : Terminator
  assymmetric filter : Subsystem
  foldback_threshold : Constant  Value=0.8
  limit_pu : Outport  VectorParamsAs1DForOutWhenUnconnected=on
  wires:
  Sum1/1 -> LPF/1(in)
  Gain/1 -> Sum2/1
  LPF/1(out) -> Gain/1
  Complex to Magnitude-Angle/1 -> assymmetric filter/1(in)
  Sum2/1 -> Saturation/1
  Constant1/1 -> Sum2/2
  foldback_threshold/1 -> Sum1/2
  Vpve_pu/1 -> Complex to Magnitude-Angle/1
  Complex to Magnitude-Angle/2 -> Terminator/1
  Saturation/1 -> limit_pu/1
  assymmetric filter/1(out) -> Sum1/1

== system My_gfm_battery_sil_1_Exciter_1/Plant controller (simplified example)/Meter ==
  note: LL RMS
  note: RMS
  note: cos x + j sin x
      | cos (x-120) + j (sin x -120)
      | cos (x+120) + j (sin x +120)
  note: cos x - j sin x
      | cos (x-120) - j (sin x -120)
      | cos (x+120) - j (sin x +120)
  note: RMS LL Pos Seq Voltage (Vd+, Vq+)
  note: vd = sqrt(1/2)*2/3*(Va * cos x + Vb * cos (x-120) + Vc * cos (x+120))
  note: vq = sqrt(1/2)*2/3*(-Va * sin x - Vb * sin (x-120) - Vc * sin (x+120))
  v : Inport
  Complex to Real-Imag : ComplexToRealImag
  Conj : Math  Operator=conj  SaturateOnIntegerOverflow=on
  Gain : Gain  Gain=sqrt(2)
  Gain1 : Gain  Gain=1/3
  Gain2 : Gain  Gain=sqrt(3)
  PLL-analog : Subsystem
  Product3 : Product
  Real-Imag to Complex : RealImagToComplex
  Sum of Elements1 : Sum  Inputs=+
  Terminator : Terminator
  Transfer Fcn : TransferFcn  Denominator=[0.05 1]
  Transfer Fcn1 : TransferFcn  Denominator=[0.05 1]
  Vpve : Outport  VectorParamsAs1DForOutWhenUnconnected=on
  wires:
  Gain2/1 -> Vpve/1
  Gain1/1 -> Complex to Real-Imag/1
  Gain/1 -> Product3/2
  Real-Imag to Complex/1 -> Gain2/1
  Conj/1 -> Gain/1
  PLL-analog/2(osc) -> Conj/1
  Complex to Real-Imag/1 -> Transfer Fcn/1
  v/1 -> Product3/1, PLL-analog/1(ref)
  Complex to Real-Imag/2 -> Transfer Fcn1/1
  Product3/1 -> Sum of Elements1/1
  Transfer Fcn/1 -> Real-Imag to Complex/1
  Sum of Elements1/1 -> Gain1/1
  Transfer Fcn1/1 -> Real-Imag to Complex/2
  PLL-analog/1(freq) -> Terminator/1

== system My_gfm_battery_sil_1_Exciter_1/Plant controller (simplified example)/VoltVAr ==
  Vpve_pu : Inport
  Abs : Abs
  Constant1 : Constant
  Gain : Gain
  LPF : Subsystem
  LPF1 : Subsystem  Commented=on
  Saturation : Saturate
  Sum1 : Sum  Inputs=|+-
  Q : Outport  VectorParamsAs1DForOutWhenUnconnected=on
  wires:
  LPF/1(out) -> Q/1
  Saturation/1 -> LPF/1(in)
  Vpve_pu/1 -> Abs/1
  Abs/1 -> Sum1/2
  Constant1/1 -> Sum1/1
  Sum1/1 -> Gain/1
  Gain/1 -> Saturation/1

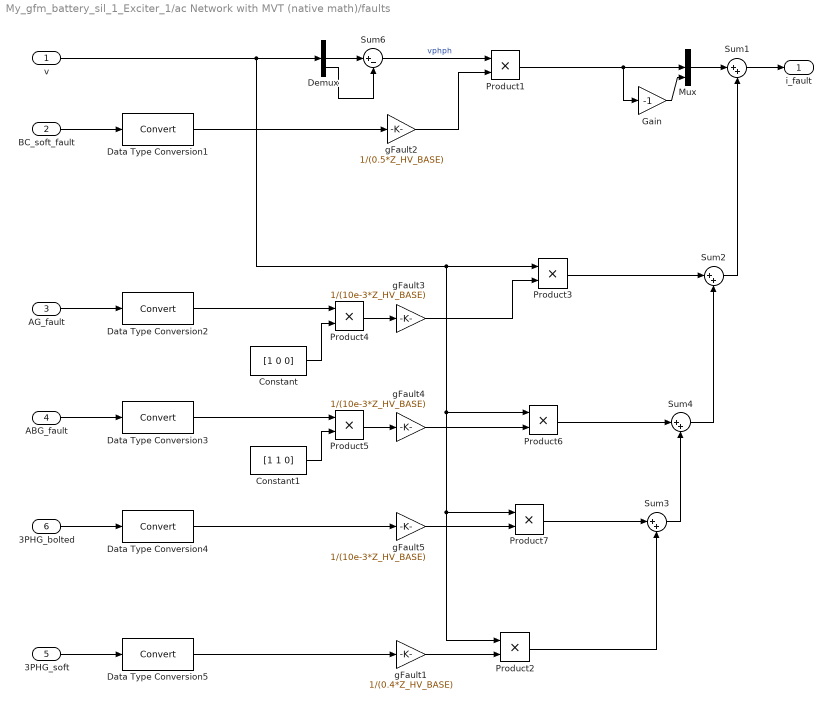
== system My_gfm_battery_sil_1_Exciter_1/ac Network with MVT (native math)/faults ==
  v : Inport
  BC_soft_fault : Inport  Port=2
  AG_fault : Inport  Port=3
  ABG_fault : Inport  Port=4
  3PHG_soft : Inport  Port=5
  3PHG_bolted : Inport  Port=6
  Constant : Constant  Value=[1 0 0]
  Constant1 : Constant  Value=[1 1 0]
  Data Type Conversion{1..5} (5 alike) : DataTypeConversion
  Demux : Demux  Outputs=3
  Gain : Gain  Gain=-1
  Mux : Mux  Inputs=3
  Product{1..7} (7 alike) : Product
  Sum{1..4} (4 alike) : Sum  Inputs=|++
  Sum6 : Sum  Inputs=|+-
  gFault1 : Gain  Gain=1/(0.4*Z_HV_BASE)
  gFault2 : Gain  Gain=1/(0.5*Z_HV_BASE)
  gFault3 : Gain  Gain=1/(10e-3*Z_HV_BASE)
  gFault4 : Gain  Gain=1/(10e-3*Z_HV_BASE)
  gFault5 : Gain  Gain=1/(10e-3*Z_HV_BASE)
  i_fault : Outport  VectorParamsAs1DForOutWhenUnconnected=on
  wires:
  Product2/1 -> Sum3/2
  gFault1/1 -> Product2/2
  Sum1/1 -> i_fault/1
  Product1/1 -> Gain/1, Mux/2
  v/1 -> Demux/1, Product3/1, Product6/1, Product7/1, Product2/1
  Demux/3 -> Sum6/2
  Demux/2 -> Sum6/1
  Gain/1 -> Mux/3
  Sum6/1 -> Product1/1  "vphph"
  gFault2/1 -> Product1/2
  gFault3/1 -> Product3/2
  Mux/1 -> Sum1/1
  Product4/1 -> gFault3/1
  Constant/1 -> Product4/2
  Constant1/1 -> Product5/2
  Product5/1 -> gFault4/1
  Product3/1 -> Sum2/1
  gFault4/1 -> Product6/2
  gFault5/1 -> Product7/2
  BC_soft_fault/1 -> Data Type Conversion1/1
  AG_fault/1 -> Data Type Conversion2/1
  ABG_fault/1 -> Data Type Conversion3/1
  3PHG_bolted/1 -> Data Type Conversion4/1
  3PHG_soft/1 -> Data Type Conversion5/1
  Sum2/1 -> Sum1/2
  Product6/1 -> Sum4/1
  Sum4/1 -> Sum2/2
  Product7/1 -> Sum3/1
  Sum3/1 -> Sum4/2
  Data Type Conversion1/1 -> gFault2/1
  Data Type Conversion2/1 -> Product4/1
  Data Type Conversion3/1 -> Product5/1
  Data Type Conversion4/1 -> gFault5/1
  Data Type Conversion5/1 -> gFault1/1

== system My_gfm_battery_sil_1_Exciter_1/ac Network with MVT (native math)/filter_caps ==
  i : Inport
  Gain1 : Gain  Gain=1/(0.03*C_LV_BASE)
  Integrator1 : Integrator
  v : Outport  VectorParamsAs1DForOutWhenUnconnected=on
  wires:
  Gain1/1 -> Integrator1/1
  Integrator1/1 -> v/1
  i/1 -> Gain1/1

== system My_gfm_battery_sil_1_Exciter_1/ac Network with MVT (native math)/filter_inductors ==
  v : Inport
  en : Inport  Port=2
  Gain1 : Gain  Gain=1/(0.02*L_LV_BASE)
  Integrator1 : Integrator  ExternalReset=level
  NOT : Logic  Operator=NOT  IconShape=distinctive  AllPortsSameDT=off  OutDataTypeStr=boolean
  i : Outport  VectorParamsAs1DForOutWhenUnconnected=on
  wires:
  NOT/1 -> Integrator1/2
  v/1 -> Gain1/1
  Integrator1/1 -> i/1
  Gain1/1 -> Integrator1/1
  en/1 -> NOT/1

== system My_gfm_battery_sil_1_Exciter_1/ac Network with MVT (native math)/solver_LPF ==
  In1 : Inport
  Gain : Gain  Gain=1/50e-6
  Integrator1 : Integrator
  Sum1 : Sum  Inputs=|+-
  Out1 : Outport  VectorParamsAs1DForOutWhenUnconnected=on
  wires:
  Gain/1 -> Integrator1/1
  Sum1/1 -> Gain/1
  Integrator1/1 -> Out1/1, Sum1/2
  In1/1 -> Sum1/1

== system My_gfm_battery_sil_1_Exciter_1/ac Network with MVT (native math)/solver_LPF1 ==
  In1 : Inport
  Gain : Gain  Gain=1/1e-3
  Integrator1 : Integrator
  Sum1 : Sum  Inputs=|+-
  Out1 : Outport  VectorParamsAs1DForOutWhenUnconnected=on
  wires:
  In1/1 -> Sum1/1
  Integrator1/1 -> Sum1/2, Out1/1
  Sum1/1 -> Gain/1
  Gain/1 -> Integrator1/1

== system My_gfm_battery_sil_1_Exciter_1/ac Network with MVT (native math)/solver_LPF3 ==
  In1 : Inport
  Gain : Gain  Gain=1/50e-6
  Integrator1 : Integrator
  Sum1 : Sum  Inputs=|+-
  Out1 : Outport  VectorParamsAs1DForOutWhenUnconnected=on
  wires:
  Gain/1 -> Integrator1/1
  Sum1/1 -> Gain/1
  Integrator1/1 -> Out1/1, Sum1/2
  In1/1 -> Sum1/1

== system My_gfm_battery_sil_1_Exciter_1/AcMeter1/PLL_3ph/SOGI ==
  in : Inport
  fnom : Inport  Port=2
  2pi : Gain  Gain=2*pi
  Integrator2 : Integrator
  Integrator3 : Integrator
  Product : Product
  Product1 : Product
  Sum4 : Sum  Inputs=|+-
  Sum5 : Sum  Inputs=|+-
  alpha : Gain  Gain=0.1
  notch : Outport  VectorParamsAs1DForOutWhenUnconnected=on
  bpf : Outport  Port=2  VectorParamsAs1DForOutWhenUnconnected=on
  wires:
  in/1 -> Sum5/1
  fnom/1 -> 2pi/1
  Integrator2/1 -> Product1/1, Sum5/2, bpf/1
  alpha/1 -> Sum4/1
  Sum5/1 -> alpha/1, notch/1
  Sum4/1 -> Product/1
  Integrator3/1 -> Sum4/2
  2pi/1 -> Product1/2, Product/2
  Product/1 -> Integrator2/1
  Product1/1 -> Integrator3/1

== system My_gfm_battery_sil_1_Exciter_1/AcMeter1/PLL_3ph/oscillator_3ph ==
  f : Inport
  Cos : Trigonometry  Operator=cos
  Gain : Gain  Gain=2*pi
  Integrator : Integrator
  Real-Imag to Complex : RealImagToComplex
  Sin : Trigonometry
  Sum1 : Sum  Inputs=|++
  phase_shift : Constant  Value=[0 -1/3 -2/3]
  osc[3] : Outport  VectorParamsAs1DForOutWhenUnconnected=on
  wires:
  f/1 -> Integrator/1
  Real-Imag to Complex/1 -> osc[3]/1
  Cos/1 -> Real-Imag to Complex/1
  Gain/1 -> Cos/1, Sin/1
  Integrator/1 -> Sum1/1
  Sin/1 -> Real-Imag to Complex/2
  phase_shift/1 -> Sum1/2
  Sum1/1 -> Gain/1

== system My_gfm_battery_sil_1_Exciter_1/AcMeter1/phasor_analysis/complex_LPF1 ==
  In1 : Inport
  Complex to Real-Imag : ComplexToRealImag
  Integrator : Integrator
  Integrator1 : Integrator
  Real-Imag to Complex : RealImagToComplex
  Sum1 : Sum  Inputs=|+-
  Sum2 : Sum  Inputs=|+-
  wLPF : Gain  Gain=wLPF
  wLPF1 : Gain  Gain=wLPF
  1 : Outport  VectorParamsAs1DForOutWhenUnconnected=on
  wires:
  Complex to Real-Imag/2 -> Sum2/1
  Sum2/1 -> wLPF1/1
  wLPF1/1 -> Integrator1/1
  Integrator1/1 -> Sum2/2, Real-Imag to Complex/2
  Real-Imag to Complex/1 -> 1/1
  In1/1 -> Complex to Real-Imag/1
  Integrator/1 -> Real-Imag to Complex/1, Sum1/2
  wLPF/1 -> Integrator/1
  Sum1/1 -> wLPF/1
  Complex to Real-Imag/1 -> Sum1/1

== system My_gfm_battery_sil_1_Exciter_1/AcMeter1/phasor_analysis1/complex_LPF1 ==
  In1 : Inport
  Complex to Real-Imag : ComplexToRealImag
  Integrator : Integrator
  Integrator1 : Integrator
  Real-Imag to Complex : RealImagToComplex
  Sum1 : Sum  Inputs=|+-
  Sum2 : Sum  Inputs=|+-
  wLPF : Gain  Gain=wLPF
  wLPF1 : Gain  Gain=wLPF
  1 : Outport  VectorParamsAs1DForOutWhenUnconnected=on
  wires:
  Complex to Real-Imag/2 -> Sum2/1
  Sum2/1 -> wLPF1/1
  wLPF1/1 -> Integrator1/1
  Integrator1/1 -> Sum2/2, Real-Imag to Complex/2
  Real-Imag to Complex/1 -> 1/1
  In1/1 -> Complex to Real-Imag/1
  Integrator/1 -> Real-Imag to Complex/1, Sum1/2
  wLPF/1 -> Integrator/1
  Sum1/1 -> wLPF/1
  Complex to Real-Imag/1 -> Sum1/1

== system My_gfm_battery_sil_1_Exciter_1/My Inverter Controller /My_acChecks_A_V2/Assert Timer ==
  note: Min one sample delay on Rise
  note: Max one sample delay on Fall
  in : Inport
  Constant : Constant  Value=T_STEP
  Constant1 : Constant  Value=0
  Constant2 : Constant  Value=TIMEOUT
  Constant3 : Constant  Value=T_STEP
  Gain : Gain  Gain=0
  Min1 : MinMax  Function=max  Inputs=2
  Min2 : MinMax  Inputs=2
  Relational Operator : RelationalOperator  Operator=>  OutDataTypeStr=boolean  RndMeth=Simplest
  Sum1 : Sum  Inputs=|++
  Sum2 : Sum  Inputs=|++
  Switch : Switch  Criteria=u2 > Threshold
  Unit Delay : UnitDelay  SampleTime=T_STEP
  out : Outport  VectorParamsAs1DForOutWhenUnconnected=on
  wires:
  Sum2/1 -> Relational Operator/1, Min2/1
  Sum1/1 -> Min2/2, Relational Operator/2
  Constant/1 -> Sum2/1
  Min2/1 -> Switch/1
  Constant1/1 -> Switch/3
  Unit Delay/1 -> Sum2/2
  in/1 -> Switch/2
  Switch/1 -> Unit Delay/1
  Relational Operator/1 -> out/1
  Min1/1 -> Sum1/1
  Constant2/1 -> Min1/1
  Constant3/1 -> Min1/2, Gain/1
  Gain/1 -> Sum1/2

== system My_gfm_battery_sil_1_Exciter_1/My Inverter Controller /My_acChecks_A_V2/Clear Timer1 ==
  note: Max one sample delay on Rise
  note: Min one sample delay on Fall
  in : Inport
  Constant : Constant  Value=T_STEP
  Constant1 : Constant  Value=0
  Constant2 : Constant  Value=TIMEOUT
  Constant3 : Constant  Value=T_STEP
  Min1 : MinMax  Function=max  Inputs=2
  Min2 : MinMax  Function=max  Inputs=2
  Relational Operator : RelationalOperator  Operator=>  OutDataTypeStr=boolean  RndMeth=Simplest
  Sum1 : Sum  Inputs=|++
  Sum2 : Sum  Inputs=|-+
  Switch : Switch  Criteria=u2 > Threshold
  Unit Delay : UnitDelay  InitialCondition=TIMER_INIT  SampleTime=T_STEP
  out : Outport  VectorParamsAs1DForOutWhenUnconnected=on
  wires:
  Sum1/1 -> Switch/1
  Sum2/1 -> Relational Operator/1, Min2/1
  Constant/1 -> Sum2/1
  Min2/1 -> Switch/3
  Constant1/1 -> Min2/2, Relational Operator/2
  Unit Delay/1 -> Sum2/2
  in/1 -> Switch/2
  Switch/1 -> Unit Delay/1
  Relational Operator/1 -> out/1
  Constant2/1 -> Min1/1
  Constant3/1 -> Min1/2, Sum1/2
  Min1/1 -> Sum1/1

== system My_gfm_battery_sil_1_Exciter_1/My Inverter Controller /My_acChecks_A_V2/Clear Timer10 ==
  note: Max one sample delay on Rise
  note: Min one sample delay on Fall
  in : Inport
  Constant : Constant  Value=T_STEP
  Constant1 : Constant  Value=0
  Constant2 : Constant  Value=TIMEOUT
  Constant3 : Constant  Value=T_STEP
  Min1 : MinMax  Function=max  Inputs=2
  Min2 : MinMax  Function=max  Inputs=2
  Relational Operator : RelationalOperator  Operator=>  OutDataTypeStr=boolean  RndMeth=Simplest
  Sum1 : Sum  Inputs=|++
  Sum2 : Sum  Inputs=|-+
  Switch : Switch  Criteria=u2 > Threshold
  Unit Delay : UnitDelay  InitialCondition=TIMER_INIT  SampleTime=T_STEP
  out : Outport  VectorParamsAs1DForOutWhenUnconnected=on
  wires:
  Sum1/1 -> Switch/1
  Sum2/1 -> Relational Operator/1, Min2/1
  Constant/1 -> Sum2/1
  Min2/1 -> Switch/3
  Constant1/1 -> Min2/2, Relational Operator/2
  Unit Delay/1 -> Sum2/2
  in/1 -> Switch/2
  Switch/1 -> Unit Delay/1
  Relational Operator/1 -> out/1
  Constant2/1 -> Min1/1
  Constant3/1 -> Min1/2, Sum1/2
  Min1/1 -> Sum1/1

== system My_gfm_battery_sil_1_Exciter_1/My Inverter Controller /My_acChecks_A_V2/Clear Timer11 ==
  note: Max one sample delay on Rise
  note: Min one sample delay on Fall
  in : Inport
  Constant : Constant  Value=T_STEP
  Constant1 : Constant  Value=0
  Constant2 : Constant  Value=TIMEOUT
  Constant3 : Constant  Value=T_STEP
  Min1 : MinMax  Function=max  Inputs=2
  Min2 : MinMax  Function=max  Inputs=2
  Relational Operator : RelationalOperator  Operator=>  OutDataTypeStr=boolean  RndMeth=Simplest
  Sum1 : Sum  Inputs=|++
  Sum2 : Sum  Inputs=|-+
  Switch : Switch  Criteria=u2 > Threshold
  Unit Delay : UnitDelay  InitialCondition=TIMER_INIT  SampleTime=T_STEP
  out : Outport  VectorParamsAs1DForOutWhenUnconnected=on
  wires:
  Sum1/1 -> Switch/1
  Sum2/1 -> Relational Operator/1, Min2/1
  Constant/1 -> Sum2/1
  Min2/1 -> Switch/3
  Constant1/1 -> Min2/2, Relational Operator/2
  Unit Delay/1 -> Sum2/2
  in/1 -> Switch/2
  Switch/1 -> Unit Delay/1
  Relational Operator/1 -> out/1
  Constant2/1 -> Min1/1
  Constant3/1 -> Min1/2, Sum1/2
  Min1/1 -> Sum1/1

== system My_gfm_battery_sil_1_Exciter_1/My Inverter Controller /My_acChecks_A_V2/Clear Timer12 ==
  note: Max one sample delay on Rise
  note: Min one sample delay on Fall
  in : Inport
  Constant : Constant  Value=T_STEP
  Constant1 : Constant  Value=0
  Constant2 : Constant  Value=TIMEOUT
  Constant3 : Constant  Value=T_STEP
  Min1 : MinMax  Function=max  Inputs=2
  Min2 : MinMax  Function=max  Inputs=2
  Relational Operator : RelationalOperator  Operator=>  OutDataTypeStr=boolean  RndMeth=Simplest
  Sum1 : Sum  Inputs=|++
  Sum2 : Sum  Inputs=|-+
  Switch : Switch  Criteria=u2 > Threshold
  Unit Delay : UnitDelay  InitialCondition=TIMER_INIT  SampleTime=T_STEP
  out : Outport  VectorParamsAs1DForOutWhenUnconnected=on
  wires:
  Sum1/1 -> Switch/1
  Sum2/1 -> Relational Operator/1, Min2/1
  Constant/1 -> Sum2/1
  Min2/1 -> Switch/3
  Constant1/1 -> Min2/2, Relational Operator/2
  Unit Delay/1 -> Sum2/2
  in/1 -> Switch/2
  Switch/1 -> Unit Delay/1
  Relational Operator/1 -> out/1
  Constant2/1 -> Min1/1
  Constant3/1 -> Min1/2, Sum1/2
  Min1/1 -> Sum1/1

== system My_gfm_battery_sil_1_Exciter_1/My Inverter Controller /My_acChecks_A_V2/Clear Timer13 ==
  note: Max one sample delay on Rise
  note: Min one sample delay on Fall
  in : Inport
  Constant : Constant  Value=T_STEP
  Constant1 : Constant  Value=0
  Constant2 : Constant  Value=TIMEOUT
  Constant3 : Constant  Value=T_STEP
  Min1 : MinMax  Function=max  Inputs=2
  Min2 : MinMax  Function=max  Inputs=2
  Relational Operator : RelationalOperator  Operator=>  OutDataTypeStr=boolean  RndMeth=Simplest
  Sum1 : Sum  Inputs=|++
  Sum2 : Sum  Inputs=|-+
  Switch : Switch  Criteria=u2 > Threshold
  Unit Delay : UnitDelay  InitialCondition=TIMER_INIT  SampleTime=T_STEP
  out : Outport  VectorParamsAs1DForOutWhenUnconnected=on
  wires:
  Sum1/1 -> Switch/1
  Sum2/1 -> Relational Operator/1, Min2/1
  Constant/1 -> Sum2/1
  Min2/1 -> Switch/3
  Constant1/1 -> Min2/2, Relational Operator/2
  Unit Delay/1 -> Sum2/2
  in/1 -> Switch/2
  Switch/1 -> Unit Delay/1
  Relational Operator/1 -> out/1
  Constant2/1 -> Min1/1
  Constant3/1 -> Min1/2, Sum1/2
  Min1/1 -> Sum1/1

== system My_gfm_battery_sil_1_Exciter_1/My Inverter Controller /My_acChecks_A_V2/Clear Timer14 ==
  note: Max one sample delay on Rise
  note: Min one sample delay on Fall
  in : Inport
  Constant : Constant  Value=T_STEP
  Constant1 : Constant  Value=0
  Constant2 : Constant  Value=TIMEOUT
  Constant3 : Constant  Value=T_STEP
  Min1 : MinMax  Function=max  Inputs=2
  Min2 : MinMax  Function=max  Inputs=2
  Relational Operator : RelationalOperator  Operator=>  OutDataTypeStr=boolean  RndMeth=Simplest
  Sum1 : Sum  Inputs=|++
  Sum2 : Sum  Inputs=|-+
  Switch : Switch  Criteria=u2 > Threshold
  Unit Delay : UnitDelay  InitialCondition=TIMER_INIT  SampleTime=T_STEP
  out : Outport  VectorParamsAs1DForOutWhenUnconnected=on
  wires:
  Sum1/1 -> Switch/1
  Sum2/1 -> Relational Operator/1, Min2/1
  Constant/1 -> Sum2/1
  Min2/1 -> Switch/3
  Constant1/1 -> Min2/2, Relational Operator/2
  Unit Delay/1 -> Sum2/2
  in/1 -> Switch/2
  Switch/1 -> Unit Delay/1
  Relational Operator/1 -> out/1
  Constant2/1 -> Min1/1
  Constant3/1 -> Min1/2, Sum1/2
  Min1/1 -> Sum1/1
